simulink model "RLSS_Logical"  (R2024b)
settings: Solver=VariableStepAuto  StartTime=0.0  StopTime=10.0  RelTol=1e-3
settings Model: Creator=Sadia Dina  LastModifiedBy=Sadia Dina

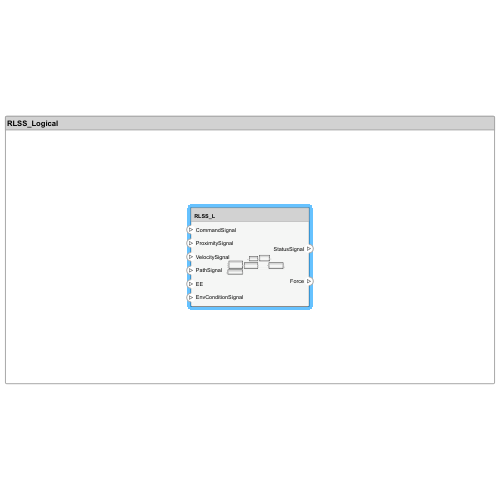
[thumbnail: Simulink's stored preview of the top-level diagram]
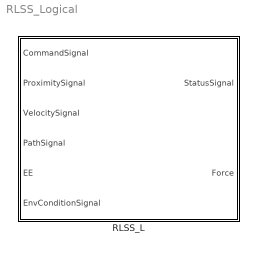
== system RLSS_Logical ==
  RLSS_L : Subsystem
      settings: PortSchema="{\"entries\":[{\"content\":{\"headerSize\":26,\"margin\":15,\"minimumSpacing\":25,\"sides\":[{\"content\":{\"connectorIds\":[\"In1\",\"In2\",\"In3\",\"In4\",\"In5\",\"In6\"]},\"type\":\"ConnectorPlacement.EquallySpacedRectSide\",\"uuid\":\"0e4af77a-90a9-4684-8ac4-a4b6cbc7152a\"},{\"content\":{\"connectorIds\":[\"Out1\",\"Out2\"],\"side\":\"RIGHT\"},\"type\":\"ConnectorPlacement.EquallySpacedRectSide\",\"uuid\":\"aea4d113-8d19-4a11-8a7a-403461391653\"},{\"content\":{\"side\":\"TOP\"},\"type\":\"ConnectorPlacement.EquallySpacedRectSide\",\"uuid\":\"fac91644-aa49-47b2-b805-0dea4a5ff633\"}]},\"type\":\"ConnectorPlacement.EquallySpacedConnector\",\"uuid\":\"0a4b06d2-cdbe-40cc-baaa-fb267f4742e4\"}],\"packageUris\":[\"http://schema.mathworks.com/mf0/Connector/R2020b\"],\"version\":\"1.0\"}"

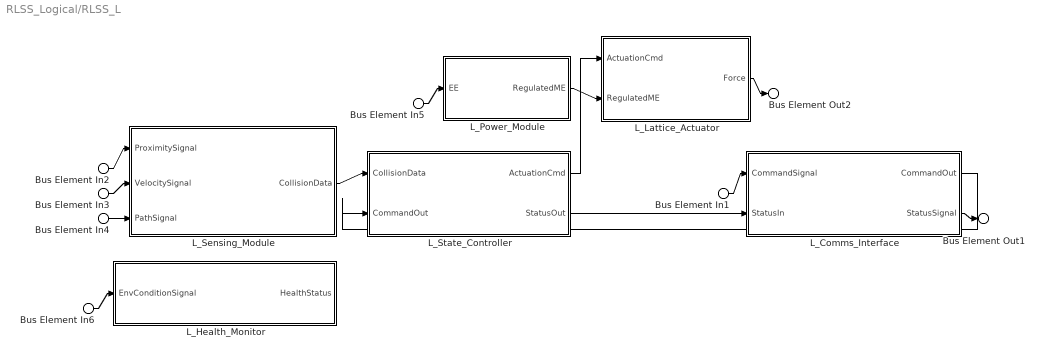
== system RLSS_Logical/RLSS_L ==
  Bus Element In1 : Inport  PortName=CommandSignal
  Bus Element In2 : Inport  Port=2  PortName=ProximitySignal
  Bus Element In3 : Inport  Port=3  PortName=VelocitySignal
  Bus Element In4 : Inport  Port=4  PortName=PathSignal
  Bus Element In5 : Inport  Port=5  PortName=EE
  Bus Element In6 : Inport  Port=6  PortName=EnvConditionSignal
  L_Comms_Interface : Subsystem
      settings: PortSchema="{\"entries\":[{\"content\":{\"headerSize\":26,\"margin\":15,\"minimumSpacing\":25,\"sides\":[{\"content\":{\"connectorIds\":[\"In1\",\"In2\"]},\"type\":\"ConnectorPlacement.EquallySpacedRectSide\",\"uuid\":\"0e4af77a-90a9-4684-8ac4-a4b6cbc7152a\"},{\"content\":{\"connectorIds\":[\"Out1\",\"Out2\"],\"side\":\"RIGHT\"},\"type\":\"ConnectorPlacement.EquallySpacedRectSide\",\"uuid\":\"aea4d113-8d19-4a11-8a7a-403461391653\"},{\"content\":{\"side\":\"TOP\"},\"type\":\"ConnectorPlacement.EquallySpacedRectSide\",\"uuid\":\"fac91644-aa49-47b2-b805-0dea4a5ff633\"}]},\"type\":\"ConnectorPlacement.EquallySpacedConnector\",\"uuid\":\"0a4b06d2-cdbe-40cc-baaa-fb267f4742e4\"}],\"packageUris\":[\"http://schema.mathworks.com/mf0/Connector/R2020b\"],\"version\":\"1.0\"}"
  L_Health_Monitor : Subsystem
      settings: PortSchema="{\"entries\":[{\"content\":{\"headerSize\":26,\"margin\":15,\"minimumSpacing\":25,\"sides\":[{\"content\":{\"connectorIds\":[\"In1\"]},\"type\":\"ConnectorPlacement.EquallySpacedRectSide\",\"uuid\":\"0e4af77a-90a9-4684-8ac4-a4b6cbc7152a\"},{\"content\":{\"connectorIds\":[\"Out1\"],\"side\":\"RIGHT\"},\"type\":\"ConnectorPlacement.EquallySpacedRectSide\",\"uuid\":\"aea4d113-8d19-4a11-8a7a-403461391653\"},{\"content\":{\"side\":\"TOP\"},\"type\":\"ConnectorPlacement.EquallySpacedRectSide\",\"uuid\":\"fac91644-aa49-47b2-b805-0dea4a5ff633\"}]},\"type\":\"ConnectorPlacement.EquallySpacedConnector\",\"uuid\":\"0a4b06d2-cdbe-40cc-baaa-fb267f4742e4\"}],\"packageUris\":[\"http://schema.mathworks.com/mf0/Connector/R2020b\"],\"version\":\"1.0\"}"
  L_Lattice_Actuator : Subsystem
      settings: PortSchema="{\"entries\":[{\"content\":{\"headerSize\":26,\"margin\":15,\"minimumSpacing\":25,\"sides\":[{\"content\":{\"connectorIds\":[\"In1\",\"In2\"]},\"type\":\"ConnectorPlacement.EquallySpacedRectSide\",\"uuid\":\"0e4af77a-90a9-4684-8ac4-a4b6cbc7152a\"},{\"content\":{\"connectorIds\":[\"Out1\"],\"side\":\"RIGHT\"},\"type\":\"ConnectorPlacement.EquallySpacedRectSide\",\"uuid\":\"aea4d113-8d19-4a11-8a7a-403461391653\"},{\"content\":{\"side\":\"TOP\"},\"type\":\"ConnectorPlacement.EquallySpacedRectSide\",\"uuid\":\"fac91644-aa49-47b2-b805-0dea4a5ff633\"}]},\"type\":\"ConnectorPlacement.EquallySpacedConnector\",\"uuid\":\"0a4b06d2-cdbe-40cc-baaa-fb267f4742e4\"}],\"packageUris\":[\"http://schema.mathworks.com/mf0/Connector/R2020b\"],\"version\":\"1.0\"}"
  L_Power_Module : Subsystem
      settings: PortSchema="{\"entries\":[{\"content\":{\"headerSize\":26,\"margin\":15,\"minimumSpacing\":25,\"sides\":[{\"content\":{\"connectorIds\":[\"In1\"]},\"type\":\"ConnectorPlacement.EquallySpacedRectSide\",\"uuid\":\"0e4af77a-90a9-4684-8ac4-a4b6cbc7152a\"},{\"content\":{\"connectorIds\":[\"Out1\"],\"side\":\"RIGHT\"},\"type\":\"ConnectorPlacement.EquallySpacedRectSide\",\"uuid\":\"aea4d113-8d19-4a11-8a7a-403461391653\"},{\"content\":{\"side\":\"TOP\"},\"type\":\"ConnectorPlacement.EquallySpacedRectSide\",\"uuid\":\"fac91644-aa49-47b2-b805-0dea4a5ff633\"}]},\"type\":\"ConnectorPlacement.EquallySpacedConnector\",\"uuid\":\"0a4b06d2-cdbe-40cc-baaa-fb267f4742e4\"}],\"packageUris\":[\"http://schema.mathworks.com/mf0/Connector/R2020b\"],\"version\":\"1.0\"}"
  L_Sensing_Module : Subsystem
      settings: PortSchema="{\"entries\":[{\"content\":{\"headerSize\":26,\"margin\":15,\"minimumSpacing\":25,\"sides\":[{\"content\":{\"connectorIds\":[\"In1\",\"In2\",\"In3\"]},\"type\":\"ConnectorPlacement.EquallySpacedRectSide\",\"uuid\":\"0e4af77a-90a9-4684-8ac4-a4b6cbc7152a\"},{\"content\":{\"connectorIds\":[\"Out1\"],\"side\":\"RIGHT\"},\"type\":\"ConnectorPlacement.EquallySpacedRectSide\",\"uuid\":\"aea4d113-8d19-4a11-8a7a-403461391653\"},{\"content\":{\"side\":\"TOP\"},\"type\":\"ConnectorPlacement.EquallySpacedRectSide\",\"uuid\":\"fac91644-aa49-47b2-b805-0dea4a5ff633\"}]},\"type\":\"ConnectorPlacement.EquallySpacedConnector\",\"uuid\":\"0a4b06d2-cdbe-40cc-baaa-fb267f4742e4\"}],\"packageUris\":[\"http://schema.mathworks.com/mf0/Connector/R2020b\"],\"version\":\"1.0\"}"
  L_State_Controller : Subsystem
      settings: PortSchema="{\"entries\":[{\"content\":{\"headerSize\":26,\"margin\":15,\"minimumSpacing\":25,\"sides\":[{\"content\":{\"connectorIds\":[\"In1\",\"In2\"]},\"type\":\"ConnectorPlacement.EquallySpacedRectSide\",\"uuid\":\"0e4af77a-90a9-4684-8ac4-a4b6cbc7152a\"},{\"content\":{\"connectorIds\":[\"Out1\",\"Out2\"],\"side\":\"RIGHT\"},\"type\":\"ConnectorPlacement.EquallySpacedRectSide\",\"uuid\":\"aea4d113-8d19-4a11-8a7a-403461391653\"},{\"content\":{\"side\":\"TOP\"},\"type\":\"ConnectorPlacement.EquallySpacedRectSide\",\"uuid\":\"fac91644-aa49-47b2-b805-0dea4a5ff633\"}]},\"type\":\"ConnectorPlacement.EquallySpacedConnector\",\"uuid\":\"0a4b06d2-cdbe-40cc-baaa-fb267f4742e4\"}],\"packageUris\":[\"http://schema.mathworks.com/mf0/Connector/R2020b\"],\"version\":\"1.0\"}"
  Bus Element Out1 : Outport  PortName=StatusSignal
  Bus Element Out2 : Outport  Port=2  PortName=Force
  wires:
  L_Sensing_Module/1(CollisionData) -> L_State_Controller/1(CollisionData)
  L_Comms_Interface/1(CommandOut) -> L_State_Controller/2(CommandOut)
  L_State_Controller/2(StatusOut) -> L_Comms_Interface/2(StatusIn)
  L_State_Controller/1(ActuationCmd) -> L_Lattice_Actuator/1(ActuationCmd)
  L_Power_Module/1(RegulatedME) -> L_Lattice_Actuator/2(RegulatedME)
  Bus Element In1/1 -> L_Comms_Interface/1(CommandSignal)
  Bus Element In2/1 -> L_Sensing_Module/1(ProximitySignal)
  Bus Element In3/1 -> L_Sensing_Module/2(VelocitySignal)
  Bus Element In4/1 -> L_Sensing_Module/3(PathSignal)
  Bus Element In5/1 -> L_Power_Module/1(EE)
  Bus Element In6/1 -> L_Health_Monitor/1(EnvConditionSignal)
  L_Comms_Interface/2(StatusSignal) -> Bus Element Out1/1
  L_Lattice_Actuator/1(Force) -> Bus Element Out2/1

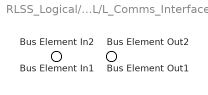
== system RLSS_Logical/RLSS_L/L_Comms_Interface ==
  Bus Element In1 : Inport  PortName=CommandSignal
  Bus Element In2 : Inport  Port=2  PortName=StatusIn
  Bus Element Out1 : Outport  PortName=CommandOut
  Bus Element Out2 : Outport  Port=2  PortName=StatusSignal

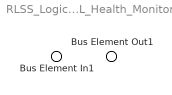
== system RLSS_Logical/RLSS_L/L_Health_Monitor ==
  Bus Element In1 : Inport  PortName=EnvConditionSignal
  Bus Element Out1 : Outport  PortName=HealthStatus

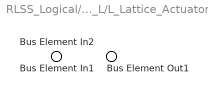
== system RLSS_Logical/RLSS_L/L_Lattice_Actuator ==
  Bus Element In1 : Inport  PortName=ActuationCmd
  Bus Element In2 : Inport  Port=2  PortName=RegulatedME
  Bus Element Out1 : Outport  PortName=Force

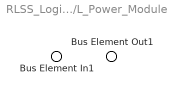
== system RLSS_Logical/RLSS_L/L_Power_Module ==
  Bus Element In1 : Inport  PortName=EE
  Bus Element Out1 : Outport  PortName=RegulatedME

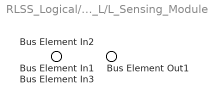
== system RLSS_Logical/RLSS_L/L_Sensing_Module ==
  Bus Element In1 : Inport  PortName=ProximitySignal
  Bus Element In2 : Inport  Port=2  PortName=VelocitySignal
  Bus Element In3 : Inport  Port=3  PortName=PathSignal
  Bus Element Out1 : Outport  PortName=CollisionData

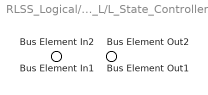
== system RLSS_Logical/RLSS_L/L_State_Controller ==
  Bus Element In1 : Inport  PortName=CollisionData
  Bus Element In2 : Inport  Port=2  PortName=CommandOut
  Bus Element Out1 : Outport  PortName=ActuationCmd
  Bus Element Out2 : Outport  Port=2  PortName=StatusOut
